simulink model "thermal_model"  (R2024b)
settings: configuration reference "MCConfiguration" (kept outside this file)
undefined symbols (not defined in the file): Ts_ThermalModel
settings Model: DataDictionary=embeddedBoard_common.sldd  Creator=ascalzo  LastModifiedBy=mfussi
settings ConfigSetRef: SourceName=MCConfiguration

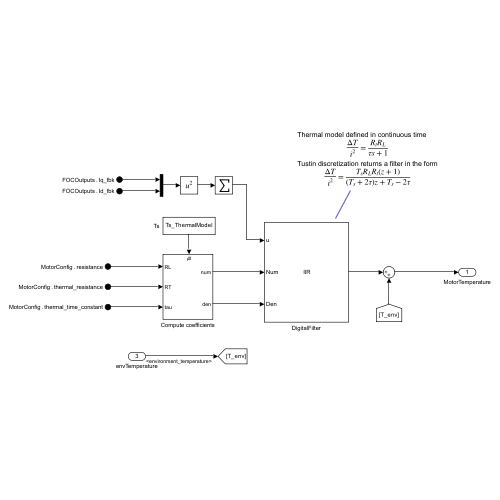
[thumbnail: Simulink's stored preview of the top-level diagram]
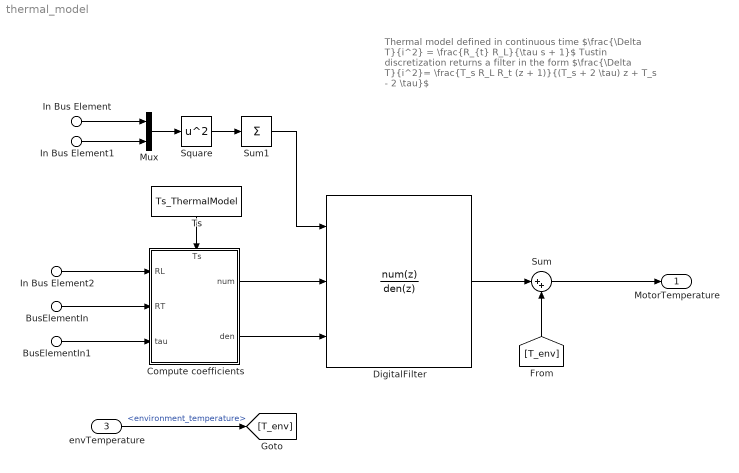
== system thermal_model ==
  note: Thermal model defined in continuous time
      | $\frac{\Delta T}{i^2} = \frac{R_{t} R_L}{\tau s + 1}$
      | Tustin discretization returns a filter in the form
      | $\frac{\Delta T}{i^2}= \frac{T_s R_L R_t (z + 1)}{(T_s + 2 \tau) z + T_s - 2 \tau}$
  In Bus Element2 : Inport  PortName=MotorConfig  Element=resistance
  BusElementIn : Inport  PortName=MotorConfig  Element=thermal_resistance
  BusElementIn1 : Inport  PortName=MotorConfig  Element=thermal_time_constant
  In Bus Element : Inport  Description=quadrature current  Port=2  PortName=FOCOutputs  Element=Iq_fbk
  In Bus Element1 : Inport  Description=direct current  Port=2  PortName=FOCOutputs  Element=Id_fbk
  envTemperature : Inport  Port=3
  Compute coefficients : Subsystem
      settings: PortSchema="{\"entries\":[{\"content\":{\"sides\":[{\"content\":{\"connectorIds\":[\"In1\",\"In2\",\"In3\"]},\"type\":\"ConnectorPlacement.EquallySpacedRectSide\",\"uuid\":\"9445c04b-443a-49eb-8603-53deaef778b1\"},{\"content\":{\"connectorIds\":[\"Out1\",\"Out2\"],\"side\":\"RIGHT\"},\"type\":\"ConnectorPlacement.EquallySpacedRectSide\",\"uuid\":\"67a2d55c-fc08-487a-81ca-c2e04bf4a356\"},{\"content\":{\"connectorIds\":[\"In4\"],\"side\":\"TOP\"},\"type\":\"ConnectorPlacement.EquallySpacedRectSide\",\"uuid\":\"bee38adf-000e-46ba-9bc9-3303aff2fd17\"}]},\"type\":\"ConnectorPlacement.EquallySpacedConnector\",\"uuid\":\"1630ff65-bc74-44ca-b473-48268a63bba7\"}],\"packageUris\":[\"http://schema.mathworks.com/mf0/Connector/R2020b\"],\"version\":\"1.0\"}"
  DigitalFilter : DiscreteFilter  NumeratorSource=Input port  Numerator="[0.02685   0.02685]"  DenominatorSource=Input port  Denominator=[1 -0.9999629]  FilterStructure=Direct form II transposed  SampleTime=Ts_ThermalModel  a0EqualsOne=on  OutDataTypeStr=Inherit: Same as input
      settings: InputPortMap=u0,p1,p3
  Mux : Mux  Inputs=2
  Square : Math  Operator=square  OutDataTypeStr=single
  Sum : Sum  Inputs=|++
  Sum1 : Sum  Inputs=+
  Ts : Constant  Value=Ts_ThermalModel  OutDataTypeStr=single  SampleTime=Ts_ThermalModel
  MotorTemperature : Outport  BusOutputAsStruct=on
  wires:
  Sum/1 -> MotorTemperature/1
  DigitalFilter/1 -> Sum/1
  BusElementIn/1 -> Compute coefficients/2(RT)
  In Bus Element2/1 -> Compute coefficients/1(RL)
  envTemperature/1 -> [T_env]  "<environment_temperature>"
  Compute coefficients/2(den) -> DigitalFilter/3
  Compute coefficients/1(num) -> DigitalFilter/2
  BusElementIn1/1 -> Compute coefficients/3(tau)
  [T_env] -> Sum/2
  Ts/1 -> Compute coefficients/4(Ts)
  Square/1 -> Sum1/1
  In Bus Element/1 -> Mux/1
  Mux/1 -> Square/1
  Sum1/1 -> DigitalFilter/1
  In Bus Element1/1 -> Mux/2

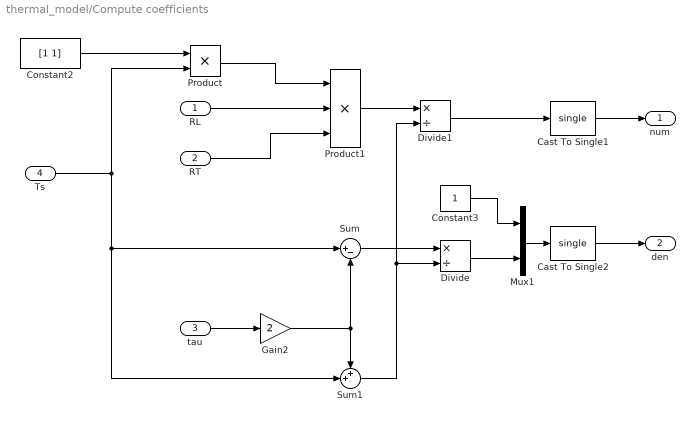
== system thermal_model/Compute coefficients ==
  RL : Inport
  RT : Inport  Port=2
  tau : Inport  Port=3
  Ts : Inport  Port=4
  Cast To Single1 : DataTypeConversion  OutDataTypeStr=single  SaturateOnIntegerOverflow=off  RndMeth=Floor
  Cast To Single2 : DataTypeConversion  OutDataTypeStr=single  SaturateOnIntegerOverflow=off  RndMeth=Floor
  Constant2 : Constant  Value=[1 1]  OutDataTypeStr=single  SampleTime=Ts_ThermalModel
  Constant3 : Constant  OutDataTypeStr=single  SampleTime=Ts_ThermalModel
  Divide : Product  Inputs=*/
  Divide1 : Product  Inputs=*/
  Gain2 : Gain  Gain=2
  Mux1 : Mux  Inputs=2
  Product : Product
  Product1 : Product  Inputs=3
  Sum : Sum  Inputs=|+-
  Sum1 : Sum  Inputs=++|
  num : Outport
  den : Outport  Port=2
  wires:
  Mux1/1 -> Cast To Single2/1
  Sum1/1 -> Divide/2, Divide1/2
  Product1/1 -> Divide1/1
  Divide1/1 -> Cast To Single1/1
  Constant2/1 -> Product/1
  tau/1 -> Gain2/1
  Constant3/1 -> Mux1/1
  RL/1 -> Product1/2
  Sum/1 -> Divide/1
  Gain2/1 -> Sum/2, Sum1/1
  Divide/1 -> Mux1/2
  Cast To Single2/1 -> den/1
  RT/1 -> Product1/3
  Cast To Single1/1 -> num/1
  Product/1 -> Product1/1
  Ts/1 -> Sum/1, Sum1/2, Product/2
